simulink model "Control_Corriente_FFB"  (R2021a)
settings: Solver=ode45  StartTime=0.0  StopTime=t_fin_control  MaxStep=Ts/50  RelTol=1e-6
InitFcn:
  | if ~exist('Kp','var') || ~exist('cmd_ws','var'), Parametros_Control; end
values from neighbouring files (symbols this model uses):
  antiwindup = 0; sim(md)    [Estabilidad_Control.m]    (also in Parametros_Control.m = 1; Verificar_Control.m = 0;')
  B = @(src,n,pos,varargin) add_block([S src],[s '/' n],'Position',pos,varargin{:})    [Crear_Modelo_Control.m]    (also in Parametros_Control.m = p_.B)
  cmd_max = 220/255    (= 0.862745098039)    [Parametros_Control.m]
  I_FS = 5    [Parametros_Control.m]
  J = p_.J    [Parametros_Control.m]
  J_eje = .01    (= 0.01)    [Figuras_Control.m]    (also in Parametros_Control.m = 0; Verificar_Control.m)
  k_acs = 0.1    [Parametros_Control.m]
  k_div = 6.8/(4.7+6.8)    (= 0.591304347826)    [Parametros_Control.m]
  Ka = p_.Ka    [Parametros_Control.m]
  Km = Ka    [Parametros_Control.m]
  Kp = Kp0*kv(j)    [Estabilidad_Control.m]    (also in Parametros_Control.m = tau_e*Ki)
  L = p_.L    [Parametros_Control.m]
  N_red = 13.7    [Parametros_Control.m]
  R = p_.R    [Parametros_Control.m]
  ruido_A = rn    [Estabilidad_Control.m]    (also in Parametros_Control.m = 0.05)
  t_adc = tau_div    (= 6.11408695652e-06)    [Parametros_Control.m]
  t_perdido = 0    [Parametros_Control.m]
  tau_div = (4.7e3*6.8e3/(4.7e3+6.8e3))*2.2e-9    (= 6.11408695652e-06)    [Parametros_Control.m]
  Tc = p_.Tc    [Parametros_Control.m]
  Ts = 1/fs    (= 5e-05)    [Parametros_Control.m]
  Ts_cmd = 2e-3    (= 0.002)    [Parametros_Control.m]
  usar_conmutado = 0; sim(md)    [Estabilidad_Control.m]    (also in Parametros_Control.m = 1)
  usar_FCEM = 0    [Parametros_Control.m]    (also in Verificar_Control.m = 1;')
  V0_acs = 2.5    [Parametros_Control.m]
  Vbus = 24    [Parametros_Control.m]
  Vmax = Dmax*Vbus    (= 20.7058823529)    [Parametros_Control.m]
undefined symbols (not defined in the file or in its folder): DiscIntNeverNeededParam, w_tc
libraries: simulink x1
settings Model: Creator=norie  LastModifiedBy=norie
settings DataIOCC: SignalLogging=off  ReturnWorkspaceOutputs=off

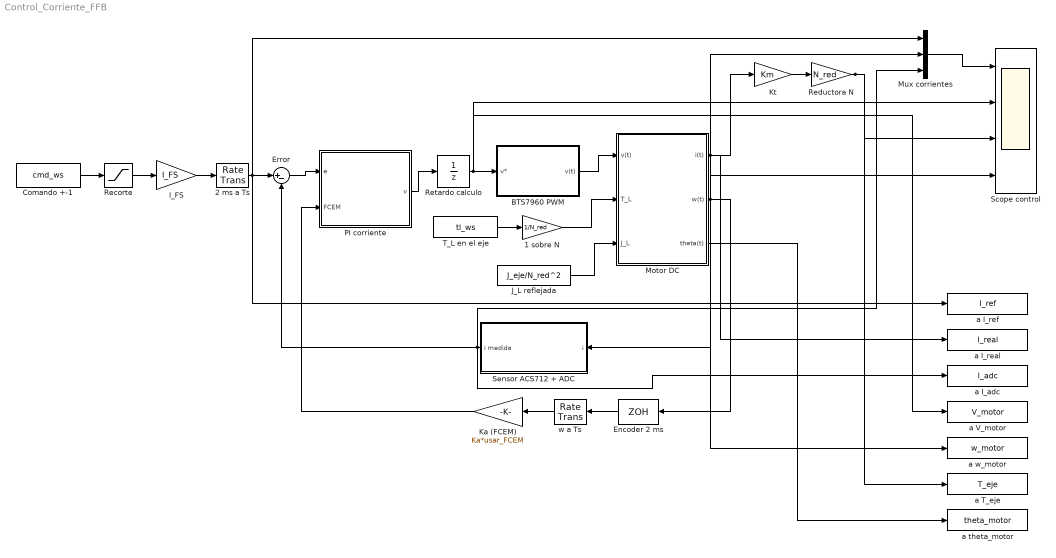
== system Control_Corriente_FFB ==
  1 sobre N : Gain  Gain=1/N_red
  2 ms a Ts : RateTransition  OutPortSampleTime=Ts
  BTS7960 PWM : Subsystem
  Comando +-1 : FromWorkspace  VariableName=cmd_ws  SampleTime=Ts_cmd  Interpolate=off  OutputAfterFinalValue=Holding final value
  Encoder 2 ms : ZeroOrderHold  SampleTime=Ts_cmd
  Error : Sum  Inputs=|+-
  I_FS : Gain  Gain=I_FS
  J_L reflejada : Constant  Value=J_eje/N_red^2
  Ka (FCEM) : Gain  Gain=Ka*usar_FCEM
  Kt : Gain  Gain=Km
  Motor DC : Subsystem
  Mux corrientes : Mux  Inputs=3
  PI corriente : Subsystem
  Recorte : Saturate  UpperLimit=cmd_max  LowerLimit=-cmd_max
  Reductora N : Gain  Gain=N_red
  Retardo calculo : UnitDelay  SampleTime=Ts  HasFrameUpgradeWarning=on
  Scope control : Scope  NumInputPorts=4
  Sensor ACS712 + ADC : Subsystem
  T_L en el eje : FromWorkspace  VariableName=tl_ws  Interpolate=off  OutputAfterFinalValue=Holding final value
  a I_adc : ToWorkspace  VariableName=I_adc  SaveFormat=Timeseries  SampleTime=-1
  a I_real : ToWorkspace  VariableName=I_real  SaveFormat=Timeseries  SampleTime=-1
  a I_ref : ToWorkspace  VariableName=I_ref  SaveFormat=Timeseries  SampleTime=-1
  a T_eje : ToWorkspace  VariableName=T_eje  SaveFormat=Timeseries  SampleTime=-1
  a V_motor : ToWorkspace  VariableName=V_motor  SaveFormat=Timeseries  SampleTime=-1
  a theta_motor : ToWorkspace  VariableName=theta_motor  SaveFormat=Timeseries  SampleTime=-1
  a w_motor : ToWorkspace  VariableName=w_motor  SaveFormat=Timeseries  SampleTime=-1
  w a Ts : RateTransition  OutPortSampleTime=Ts
  wires:
  T_L en el eje/1 -> 1 sobre N/1
  1 sobre N/1 -> Motor DC/2(T_L)
  J_L reflejada/1 -> Motor DC/3(J_L)
  Comando +-1/1 -> Recorte/1
  Recorte/1 -> I_FS/1
  I_FS/1 -> 2 ms a Ts/1
  2 ms a Ts/1 -> Error/1, Mux corrientes/1, a I_ref/1
  Error/1 -> PI corriente/1(e)
  PI corriente/1(v) -> Retardo calculo/1
  Retardo calculo/1 -> BTS7960 PWM/1(v*), Scope control/2, a V_motor/1
  BTS7960 PWM/1(v(t)) -> Motor DC/1(v(t))
  Motor DC/1(i(t)) -> Kt/1, Sensor ACS712 + ADC/1(i), Mux corrientes/2, a I_real/1
  Kt/1 -> Reductora N/1
  Sensor ACS712 + ADC/1(i medida) -> Error/2, Mux corrientes/3, a I_adc/1
  Motor DC/2(w(t)) -> Encoder 2 ms/1, Scope control/4, a w_motor/1
  Encoder 2 ms/1 -> w a Ts/1
  w a Ts/1 -> Ka (FCEM)/1
  Ka (FCEM)/1 -> PI corriente/2(FCEM)
  Mux corrientes/1 -> Scope control/1
  Reductora N/1 -> Scope control/3, a T_eje/1
  Motor DC/3(theta(t)) -> a theta_motor/1

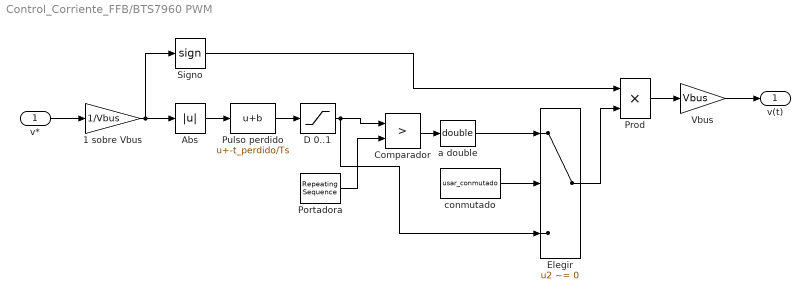
== system Control_Corriente_FFB/BTS7960 PWM ==
  v* : Inport
  1 sobre Vbus : Gain  Gain=1/Vbus
  Abs : Abs  ZeroCross=off
  Comparador : RelationalOperator  Operator=>  OutDataTypeStr=boolean  RndMeth=Simplest
  D 0..1 : Saturate  UpperLimit=1  LowerLimit=0  ZeroCross=off
  Elegir : Switch  Criteria=u2 ~= 0  ZeroCross=off
  Portadora : simulink/Sources/Repeating Sequence  rep_seq_t=[0 Ts/2-t_adc Ts-t_adc Ts]  rep_seq_y=[1-2*t_adc/Ts 0 1 1-2*t_adc/Ts]
  Prod : Product
  Pulso perdido : Bias  Bias=-t_perdido/Ts
  Signo : Signum  ZeroCross=off
  Vbus : Gain  Gain=Vbus
  a double : DataTypeConversion  OutDataTypeStr=double
  conmutado : Constant  Value=usar_conmutado
  v(t) : Outport
  wires:
  v*/1 -> 1 sobre Vbus/1
  1 sobre Vbus/1 -> Abs/1, Signo/1
  Abs/1 -> Pulso perdido/1
  Pulso perdido/1 -> D 0..1/1
  D 0..1/1 -> Comparador/1, Elegir/3
  Portadora/1 -> Comparador/2
  Comparador/1 -> a double/1
  a double/1 -> Elegir/1
  conmutado/1 -> Elegir/2
  Signo/1 -> Prod/1
  Elegir/1 -> Prod/2
  Prod/1 -> Vbus/1
  Vbus/1 -> v(t)/1

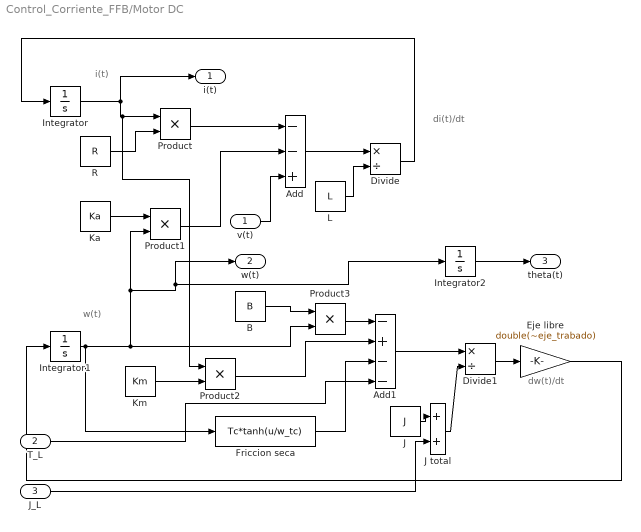
== system Control_Corriente_FFB/Motor DC ==
  note: dw(t)/dt
  note: di(t)/dt
  note: w(t)
  note: i(t)
  v(t) : Inport
  T_L : Inport  Port=2
  J_L : Inport  Port=3
  Add : Sum  Inputs=--+
  Add1 : Sum  Inputs=-+--
  B : Constant  Value=B
  Divide : Product  Inputs=*/
  Divide1 : Product  Inputs=*/
  Eje libre : Gain  Gain=double(~eje_trabado)
  Friccion seca : Fcn  Expr=Tc*tanh(u/w_tc)
  Integrator : Integrator
  Integrator1 : Integrator
  Integrator2 : Integrator
  J : Constant  Value=J
  J total : Sum
  Ka : Constant  Value=Ka
  Km : Constant  Value=Km
  L : Constant  Value=L
  Product{,1..3} (4 alike) : Product
  R : Constant  Value=R
  i(t) : Outport  VectorParamsAs1DForOutWhenUnconnected=off
  w(t) : Outport  Port=2  VectorParamsAs1DForOutWhenUnconnected=off
  theta(t) : Outport  Port=3  VectorParamsAs1DForOutWhenUnconnected=off
  wires:
  Eje libre/1 -> Integrator1/1
  Divide1/1 -> Eje libre/1
  Friccion seca/1 -> Add1/3
  Product2/1 -> Add1/2
  Km/1 -> Product2/2
  B/1 -> Product3/1
  Integrator2/1 -> theta(t)/1
  L/1 -> Divide/2
  Product/1 -> Add/1
  Add/1 -> Divide/1
  Product1/1 -> Add/2
  Product3/1 -> Add1/1
  Ka/1 -> Product1/1
  v(t)/1 -> Add/3
  Add1/1 -> Divide1/1
  R/1 -> Product/2
  Integrator1/1 -> Friccion seca/1, Product1/2, Integrator2/1, w(t)/1, Product3/2
  Integrator/1 -> Product/1, Product2/1, i(t)/1
  Divide/1 -> Integrator/1
  T_L/1 -> Add1/4
  J/1 -> J total/1
  J_L/1 -> J total/2
  J total/1 -> Divide1/2

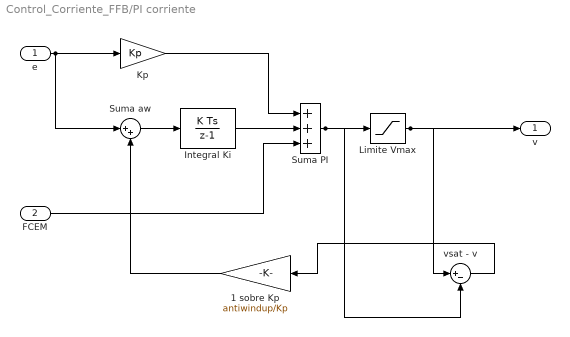
== system Control_Corriente_FFB/PI corriente ==
  e : Inport
  FCEM : Inport  Port=2
  1 sobre Kp : Gain  Gain=antiwindup/Kp
  Integral Ki : DiscreteIntegrator  gainval=Ki  SampleTime=Ts  ICPrevOutput=DiscIntNeverNeededParam  ICPrevScaledInput=DiscIntNeverNeededParam
  Kp : Gain  Gain=Kp
  Limite Vmax : Saturate  UpperLimit=Vmax  LowerLimit=-Vmax
  Suma PI : Sum  Inputs=+++
  Suma aw : Sum  Inputs=|++
  vsat - v : Sum  Inputs=|+-
  v : Outport
  wires:
  e/1 -> Kp/1, Suma aw/1
  Kp/1 -> Suma PI/1
  Suma aw/1 -> Integral Ki/1
  Integral Ki/1 -> Suma PI/2
  FCEM/1 -> Suma PI/3
  Suma PI/1 -> Limite Vmax/1, vsat - v/2
  Limite Vmax/1 -> v/1, vsat - v/1
  vsat - v/1 -> 1 sobre Kp/1
  1 sobre Kp/1 -> Suma aw/2

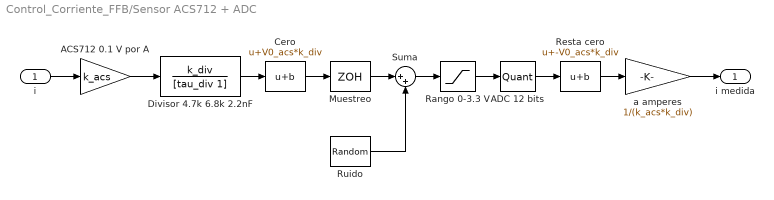
== system Control_Corriente_FFB/Sensor ACS712 + ADC ==
  i : Inport
  ACS712 0.1 V por A : Gain  Gain=k_acs
  ADC 12 bits : Quantizer  QuantizationInterval=lsb_adc
  Cero : Bias  Bias=V0_acs*k_div
  Divisor 4.7k 6.8k 2.2nF : TransferFcn  Numerator=k_div  Denominator=[tau_div 1]
  Muestreo : ZeroOrderHold  SampleTime=Ts
  Rango 0-3.3 V : Saturate  UpperLimit=3.3  LowerLimit=0
  Resta cero : Bias  Bias=-V0_acs*k_div
  Ruido : RandomNumber  Variance=(ruido_A*k_acs*k_div)^2  SampleTime=Ts
  Suma : Sum  Inputs=|++
  a amperes : Gain  Gain=1/(k_acs*k_div)
  i medida : Outport
  wires:
  i/1 -> ACS712 0.1 V por A/1
  ACS712 0.1 V por A/1 -> Divisor 4.7k 6.8k 2.2nF/1
  Divisor 4.7k 6.8k 2.2nF/1 -> Cero/1
  Cero/1 -> Muestreo/1
  Muestreo/1 -> Suma/1
  Ruido/1 -> Suma/2
  Suma/1 -> Rango 0-3.3 V/1
  Rango 0-3.3 V/1 -> ADC 12 bits/1
  ADC 12 bits/1 -> Resta cero/1
  Resta cero/1 -> a amperes/1
  a amperes/1 -> i medida/1
